simulink model "FOC"  (R2022b)
settings: Solver=FixedStepAuto  StartTime=0.0  StopTime=4  FixedStep=2e-7  RelTol=1e-3
undefined symbols (not defined in the file): sigbuilder_block
libraries: slpidlib x3, spsDCVoltageSourceLib x1, spsPermanentMagnetSynchronousMachineLib x1, simulink x1, spsUniversalBridgeLib x1, spspowerguiLib x1
settings Model: Creator=SSC  LastModifiedBy=SSC

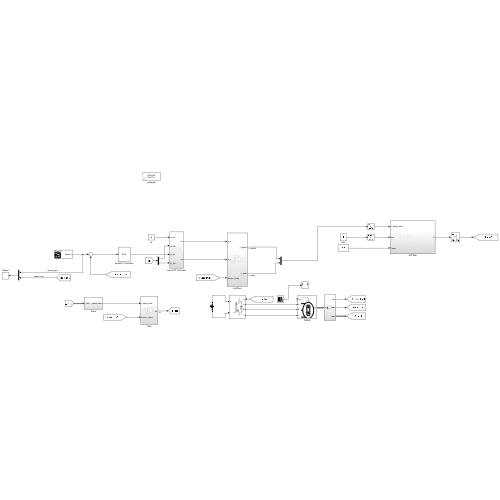
[thumbnail: Simulink's stored preview of the top-level diagram]
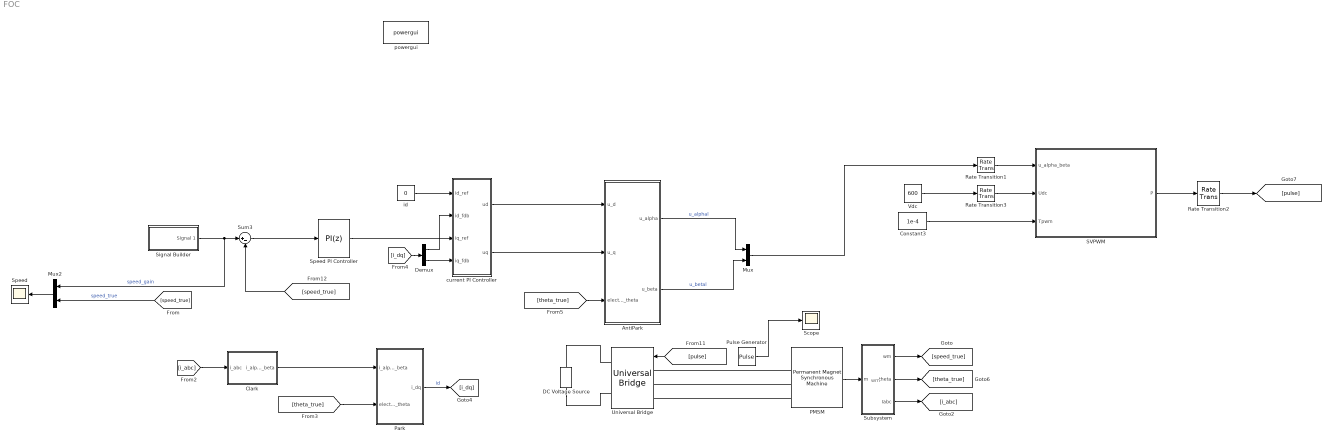
== system FOC ==
  note: wm
  AntiPark : Subsystem
  Clark : Subsystem
  Constant3 : Constant  Value=1e-4
  DC Voltage Source : spsDCVoltageSourceLib/DC Voltage Source  Amplitude=600  Measurements=None
  Demux : Demux  Outputs=2
  Mux : Mux  Inputs=2
  Mux2 : Mux  Inputs=2
  PMSM : spsPermanentMagnetSynchronousMachineLib/Permanent Magnet Synchronous Machine  NbPhases=3  FluxDistribution=Sinusoidal  RotorType=Salient-pole  MechanicalLoad=Torque Tm  PresetModel=No  ShowDetailedParameters=on  MeasurementBus=off  Resistance=0.91  Inductance=8.5e-3  dqInductances=[0.00396,0.00796]  La=8.5e-3  MachineConstant=Flux linkage established by magnets (V.s)  Flux=0.446  VoltageCst=161.7909  TorqueCst=1.338  Flat=120  Mechanical=[0.074 0.008 2 0]  PolePairs=4  InitialConditions=[0,0, 0,0]  InitialConditions5ph=[0 0 0 0 0 0]  RefAngle=Aligned with phase A axis (original Park)  IterativeDiscreteModel=Trapezoidal non iterative  TsBlock=-1  TsPowergui=0
  Park : Subsystem
  Pulse Generator : DiscretePulseGenerator  PulseType=Time based  Period=3  PulseWidth=33.3  PhaseDelay=2.5
  Rate Transition1 : RateTransition  OutPortSampleTimeOpt=Inherit
  Rate Transition2 : RateTransition
  Rate Transition3 : RateTransition  OutPortSampleTimeOpt=Inherit
  SVPWM : Subsystem
  Scope : Scope
  Signal Builder : Subsystem  Tag=STV Subsys  LoadFcn=sigbuilder_block('load');  StartFcn=sigbuilder_block('start');  StopFcn=sigbuilder_block('stop');  ClipboardFcn=sigbuilder_block('clipboard');  mask(Sigbuilder block){tuvar=[0:10]}
      mask help: Simulink:masks:SigbuilderBlock_MD
      mask init:
      | if ~strcmp(get_param(bdroot(gcbh),'SimulationStatus'),'stopped') tuvar = sigbuilder_block('maskInit'); end
      settings: CopyFcn=sigbuilder_block('copy');  DeleteFcn=sigbuilder_block('delete');  ModelCloseFcn=sigbuilder_block('modelClose');  PreSaveFcn=sigbuilder_block('preSave');  PauseFcn=sigbuilder_block('pause');  ContinueFcn=sigbuilder_block('continue');  NameChangeFcn=sigbuilder_block('namechange');  OpenFcn=sigbuilder_block('open',[290.5 134.5 550.5 400 ]);  CloseFcn=sigbuilder_block('close');
      mask Display: plot(0, 0, 100, 100,[2, 2, 32, 32, 2], [68, 8, 8, 68, 68],[32, 2], [38, 38], [32, 19, 2],[53, 60, 44], [32, 17, 17, 2],[16, 16, 31, 31]);txt = getActiveGroup(gcbh);text(2, 100, txt,'verticalAlignment', 'top');
  Speed : Scope
  Speed PI Controller : slpidlib/PID Controller  Controller=PI  Form=Parallel  TimeDomain=Discrete-time  UseExternalTs=off  SampleTime=1e-4  IntegratorMethod=Forward Euler  FilterMethod=Forward Euler  ControllerParametersSource=internal  P=3.736/30  I=44.84/30  UseKiTs=off  D=0  N=100  UseFilter=on  TunerSelectOption=Transfer Function Based (PID Tuner App)  InitialConditionSource=internal  InitialConditionForIntegrator=0  InitialConditionForFilter=0  DifferentiatorICPrevScaledInput=0  ExternalReset=none  TrackingMode=off  Kt=1  LimitOutput=off  SatLimitsSource=internal  UpperSaturationLimit=5.65  LowerSaturationLimit=-5.65  LinearizeAsGain=on  AntiWindupMode=clamping  Kb=1  LimitIntegrator=off  UpperIntegratorSaturationLimit=inf  LowerIntegratorSaturationLimit=-inf  POutMin=[]  POutMax=[]  IOutMin=[]  IOutMax=[]  DOutMin=[]  DOutMax=[]  NOutMin=[]  NOutMax=[]  SumOutMin=[]  SumOutMax=[]  SaturationOutMin=[]  SaturationOutMax=[]  PParamMin=[]  PParamMax=[]  IParamMin=[]  IParamMax=[]  DParamMin=[]  DParamMax=[]  NParamMin=[]  NParamMax=[]  KbParamMin=[]  KbParamMax=[]  KtParamMin=[]  KtParamMax=[]  KbOutMin=[]  KbOutMax=[]  KtOutMin=[]  KtOutMax=[]  IntegratorOutMin=[]  IntegratorOutMax=[]  FilterOutMin=[]  FilterOutMax=[]  SumI1OutMin=[]  SumI1OutMax=[]  SumI2OutMin=[]  SumI2OutMax=[]  SumI3OutMin=[]  SumI3OutMax=[]  SumI4OutMin=[]  SumI4OutMax=[]  SumDOutMin=[]  SumDOutMax=[]  DifferentiatorOutMin=[]  DifferentiatorOutMax=[]  FilterDiffOutCoefMin=[]  FilterDiffOutCoefMax=[]  ReciprocalOutMin=[]  ReciprocalOutMax=[]  SumDenOutMin=[]  SumDenOutMax=[]  SumNumOutMin=[]  SumNumOutMax=[]  DivideOutMin=[]  DivideOutMax=[]  UdiffTsProdOutMin=[]  UdiffTsProdOutMax=[]  NTsProdOutMin=[]  NTsProdOutMax=[]  UintegralTsProdOutMin=[]  UintegralTsProdOutMax=[]  UngainTsProdOutMin=[]  UngainTsProdOutMax=[]  ClampingZeroOutDataTypeStr=Inherit: Inherit via back propagation  ClampingZeroOutMin=[]  ClampingZeroOutMax=[]  FilterDenConstantOutDataTypeStr=Inherit: Inherit via back propagation  FilterDenConstantOutMin=[]  FilterDenConstantOutMax=[]  PCopyOutDataTypeStr=Inherit: Inherit via back propagation  PCopyOutMin=[]  PCopyOutMax=[]  NCopyOutDataTypeStr=Inherit: Inherit via back propagation  NCopyOutMin=[]  NCopyOutMax=[]  IntegratorContinuousStateAttributes=''  IntegratorStateMustResolveToSignalObject=off  IntegratorRTWStateStorageClass=Auto  FilterContinuousStateAttributes=''  FilterStateMustResolveToSignalObject=off  FilterRTWStateStorageClass=Auto  ParallelPVariant=InternalParameters  IdealPVariant=Disabled  IVariant=InternalParameters  DVariant=Disabled  IntegratorVariant=Discrete  SatVariant=Disabled  AWVariant=Passthrough  PCopyVariant=Disabled  TRVariant=Disabled  FdbkBlocksVariant=Forward  IdealPFdbkVariant=Disabled  SatFdbkVariant=Disabled  DerivativeFilterVariant=Disabled  NVariant=Disabled  NCopyVariant=Disabled_SignalSpec  FilterICVariant=Disabled  IntegratorICVariant=InternalICs  ExternalResetVariant=Disabled  TRSumVariant=Passthrough  SumFdbkVariant=Disabled  SumVariant=Sum_PI  TsampFilterVariant=InternalTs  TsampNgainVariant=Passthrough  TsampIntegralVariant=Passthrough  ExternalSaturationOutDataTypeStr=Inherit: Same as second input
  Subsystem : Subsystem
  Sum3 : Sum  Inputs=|+-
  Universal Bridge : spsUniversalBridgeLib/Universal Bridge  Arms=3  SnubberResistance=1e5  SnubberCapacitance=inf  Device=IGBT / Diodes  Ron=1e-3  Lon=0  ForwardVoltages="[  0  0  ]"  ForwardVoltage=0  GTOparameters=[ 10e-6 , 20e-6 ]  IGBTparameters=[ 1e-6 , 2e-6 ]  Measurements=None  Measurements_2=None  converterType=Rectifier
  Vdc : Constant  Value=600
  current PI Controller : Subsystem
  id : Constant  Value=0
  powergui : spspowerguiLib/powergui  Priority=1  SimulationMode=Discrete  SampleTime=2e-7  frequency=60  Iterations=50  frequencyindice=0  Pbase=100e6  ErrMax=1e-4  UnitsV=kV  UnitsW=MW  buscounter=0  FunctionMessages=off  echomessages=off  EnableUseOfTLC=off  CurrentSourceSwitches=off  DisableSnubberDevices=off  DisableRonSwitches=off  DisableVfSwitches=off  DisplayEquations=off  AutomaticDiscreteSolvers=off  SolverType=Tustin/Backward Euler (TBE)  Interpol=off  ExternalGateDelay=off  methode=off  Ts=100  x0status=blocks  SPID=on  SwTol=0  HookPort=off  NonlinearTolerance=1e-4  nMaxIteration=100  ContinueOnMaxIteration=off  RestoreLinks=warning  ResistiveCurrentMeasurement=off  Frange=[0:2:500]  Ylog=off  Xlog=on  ShowGrid=off  save=off  variable=ZData  structure=0  ZoomFFT=off  StartTime=0.0  cycles=1  DisplayStyle=1  fundamental=60  FreqAxis=off  MaxFrequency=1000  frequencyindicesteady=1  RmsSteady=1  display=off
  wires:
  [speed_true] -> Sum3/2
  Rate Transition1/1 -> SVPWM/1(u_alpha_beta)
  Demux/1 -> current PI Controller/2(id_fdb)
  Pulse Generator/1 -> Scope/1
  Speed PI Controller/1 -> current PI Controller/3(iq_ref)
  Clark/1(i_alpha_beta) -> Park/1(i_alpha_beta)
  id/1 -> current PI Controller/1(id_ref)
  [theta_true] -> Park/2(electric_theta)
  [pulse] -> Universal Bridge/1
  Demux/2 -> current PI Controller/4(iq_fdb)
  [i_dq] -> Demux/1
  Mux/1 -> Rate Transition1/1
  current PI Controller/2(uq) -> AntiPark/2(u_q)
  AntiPark/2(u_beta) -> Mux/2  "u_betal"
  Sum3/1 -> Speed PI Controller/1
  Rate Transition2/1 -> [pulse]
  Vdc/1 -> Rate Transition3/1
  Mux2/1 -> Speed/1
  Park/1(i_dq) -> [i_dq]  "id"
  Rate Transition3/1 -> SVPWM/2(Udc)
  PMSM/1 -> Subsystem/1(m)
  [theta_true] -> AntiPark/3(electric_theta)
  AntiPark/1(u_alpha) -> Mux/1  "u_alphal"
  Subsystem/1(wm) -> [speed_true]
  Constant3/1 -> SVPWM/3(Tpwm)
  Signal Builder/1(Signal 1) -> Mux2/1, Sum3/1  "speed_gain"
  current PI Controller/1(ud) -> AntiPark/1(u_d)
  Subsystem/3(Iabc) -> [i_abc]
  [speed_true] -> Mux2/2  "speed_true"
  SVPWM/1(P) -> Rate Transition2/1
  Subsystem/2(theta) -> [theta_true]
  [i_abc] -> Clark/1(i_abc)
  connections:
  Universal Bridge/RConn1 -- DC Voltage Source/RConn1
  PMSM/LConn3 -- Universal Bridge/LConn3
  DC Voltage Source/LConn1 -- Universal Bridge/RConn2
  PMSM/LConn1 -- Universal Bridge/LConn1
  PMSM/LConn2 -- Universal Bridge/LConn2

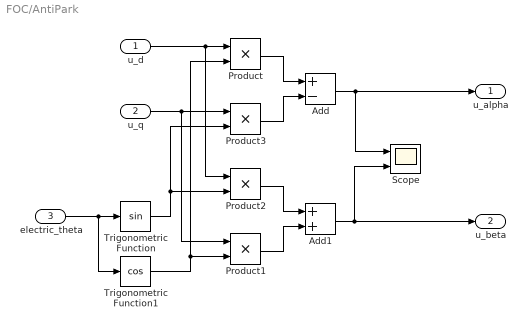
== system FOC/AntiPark ==
  u_d : Inport
  u_q : Inport  Port=2
  electric_theta : Inport  Port=3
  Add : Sum  Inputs=+-
  Add1 : Sum
  Product{,1..3} (4 alike) : Product
  Scope : Scope  NumInputPorts=2
  Trigonometric Function : Trigonometry
  Trigonometric Function1 : Trigonometry  Operator=cos
  u_alpha : Outport
  u_beta : Outport  Port=2
  wires:
  electric_theta/1 -> Trigonometric Function1/1, Trigonometric Function/1
  u_d/1 -> Product2/1, Product/1
  Trigonometric Function1/1 -> Product/2, Product1/2
  u_q/1 -> Product1/1, Product3/1
  Trigonometric Function/1 -> Product2/2, Product3/2
  Product/1 -> Add/1
  Product3/1 -> Add/2
  Add/1 -> Scope/1, u_alpha/1
  Product2/1 -> Add1/1
  Product1/1 -> Add1/2
  Add1/1 -> Scope/2, u_beta/1

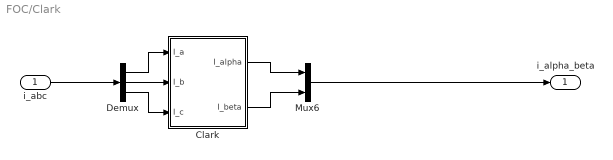
== system FOC/Clark ==
  i_abc : Inport
  Clark : Subsystem
  Demux : Demux  Outputs=3
  Mux6 : Mux  Inputs=2
  i_alpha_beta : Outport  VectorParamsAs1DForOutWhenUnconnected=off
  wires:
  Clark/2(I_beta) -> Mux6/2
  Mux6/1 -> i_alpha_beta/1
  Demux/3 -> Clark/3(I_c)
  Clark/1(I_alpha) -> Mux6/1
  i_abc/1 -> Demux/1
  Demux/2 -> Clark/2(I_b)
  Demux/1 -> Clark/1(I_a)

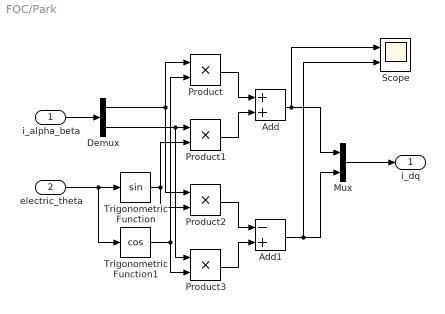
== system FOC/Park ==
  i_alpha_beta : Inport
  electric_theta : Inport  Port=2
  Add : Sum
  Add1 : Sum  Inputs=-+
  Demux : Demux  Outputs=2
  Mux : Mux  Inputs=2
  Product{,1..3} (4 alike) : Product
  Scope : Scope  NumInputPorts=2
  Trigonometric Function : Trigonometry
  Trigonometric Function1 : Trigonometry  Operator=cos
  i_dq : Outport
  wires:
  electric_theta/1 -> Trigonometric Function1/1, Trigonometric Function/1
  Trigonometric Function1/1 -> Product3/2, Product/2
  Demux/2 -> Product3/1, Product1/1
  Trigonometric Function/1 -> Product2/2, Product1/2
  Product/1 -> Add/1
  Product1/1 -> Add/2
  Product2/1 -> Add1/1
  Product3/1 -> Add1/2
  Add/1 -> Scope/1, Mux/1
  Add1/1 -> Scope/2, Mux/2
  Demux/1 -> Product/1, Product2/1
  i_alpha_beta/1 -> Demux/1
  Mux/1 -> i_dq/1

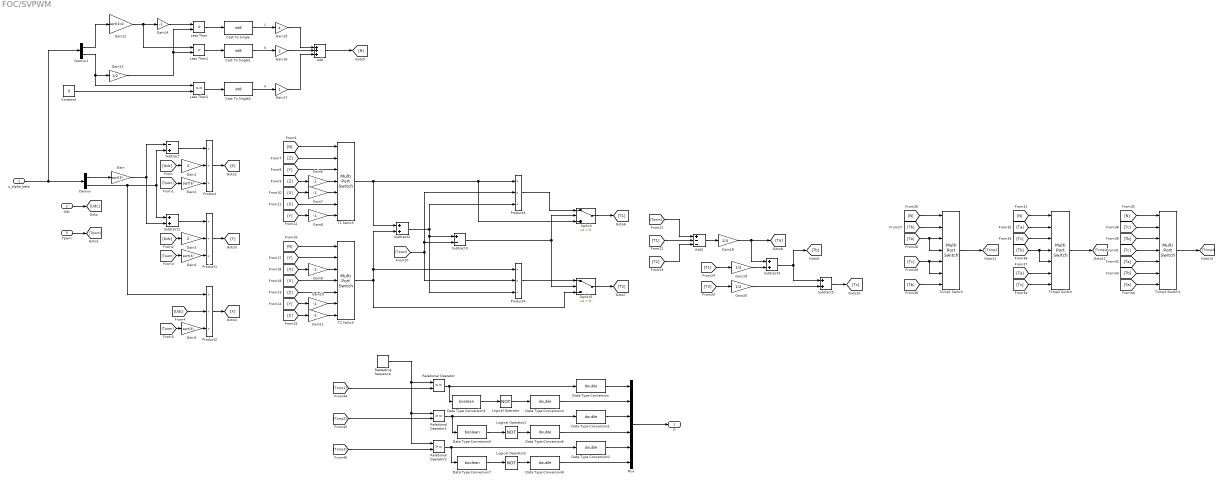
== system FOC/SVPWM ==
  u_alpha_beta : Inport
  Udc : Inport  Port=2
  Tpwm : Inport  Port=3
  Add : Sum  Inputs=+++
  Add1 : Sum  Inputs=+--
  Cast To Single : DataTypeConversion  OutDataTypeStr=int8  SaturateOnIntegerOverflow=off  RndMeth=Floor
  Cast To Single1 : DataTypeConversion  OutDataTypeStr=int8  SaturateOnIntegerOverflow=off  RndMeth=Floor
  Cast To Single2 : DataTypeConversion  OutDataTypeStr=int8  SaturateOnIntegerOverflow=off  RndMeth=Floor
  Constant : Constant  Value=0
  Data Type Conversion{,1..2,4,6,8} (6 alike) : DataTypeConversion  OutDataTypeStr=double  SaturateOnIntegerOverflow=off  RndMeth=Floor
  Data Type Conversion3 : DataTypeConversion  OutDataTypeStr=boolean  SaturateOnIntegerOverflow=off  RndMeth=Floor
  Data Type Conversion5 : DataTypeConversion  OutDataTypeStr=boolean  SaturateOnIntegerOverflow=off  RndMeth=Floor
  Data Type Conversion7 : DataTypeConversion  OutDataTypeStr=boolean  SaturateOnIntegerOverflow=off  RndMeth=Floor
  Demux : Demux  Outputs=2
  Demux1 : Demux  Outputs=2
  Gain{,2,4..5} (4 alike) : Gain  Gain=sqrt(3)
  Gain1 : Gain  Gain=2
  Gain{6..11,14} (7 alike) : Gain  Gain=-1
  Gain12 : Gain  Gain=sqrt(3)/2
  Gain13 : Gain  Gain=1/2
  Gain15 : Gain  Gain=4
  Gain16 : Gain  Gain=2
  Gain17 : Gain
  Gain18 : Gain  Gain=1/4
  Gain19 : Gain  Gain=1/2
  Gain20 : Gain  Gain=1/2
  Gain3 : Gain  Gain=2
  Less Than : RelationalOperator  Operator=>  OutDataTypeStr=boolean  RndMeth=Simplest  InputSameDT=off
  Less Than1 : RelationalOperator  Operator=>  OutDataTypeStr=boolean  RndMeth=Simplest  InputSameDT=off
  Less Than2 : RelationalOperator  OutDataTypeStr=boolean  RndMeth=Simplest  InputSameDT=off
  Logical Operator : Logic  Operator=NOT  AllPortsSameDT=off  OutDataTypeStr=boolean
  Logical Operator1 : Logic  Operator=NOT  AllPortsSameDT=off  OutDataTypeStr=boolean
  Logical Operator2 : Logic  Operator=NOT  AllPortsSameDT=off  OutDataTypeStr=boolean
  Mux : Mux  Inputs=6
  Product : Product  Inputs=*/*
  Product1 : Product  Inputs=*/*
  Product2 : Product  Inputs=*/*
  Product3 : Product  Inputs=**/
  Product4 : Product  Inputs=**/
  Relational Operator : RelationalOperator  OutDataTypeStr=boolean  RndMeth=Simplest  InputSameDT=off
  Relational Operator1 : RelationalOperator  OutDataTypeStr=boolean  RndMeth=Simplest  InputSameDT=off
  Relational Operator2 : RelationalOperator  OutDataTypeStr=boolean  RndMeth=Simplest  InputSameDT=off
  Repeating Sequence : simulink/Sources/Repeating Sequence  rep_seq_t=[0 1e-4 2e-4]  rep_seq_y=[0 0.5e-4 0]
  Subtract : Sum  Inputs=-+
  Subtract{1..2,4..5} (4 alike) : Sum
  Subtract3 : Sum  Inputs=+-
  Switch : Switch  Criteria=u2 > Threshold  SaturateOnIntegerOverflow=off  InputSameDT=off
  Switch1 : Switch  Criteria=u2 > Threshold  SaturateOnIntegerOverflow=off  InputSameDT=off
  T1 Switch : MultiPortSwitch  Inputs=6  SaturateOnIntegerOverflow=off  InputSameDT=off
  T2 Switch : MultiPortSwitch  Inputs=6  SaturateOnIntegerOverflow=off  InputSameDT=off
  Tcmp1 Switch : MultiPortSwitch  Inputs=6  SaturateOnIntegerOverflow=off  InputSameDT=off
  Tcmp2 Switch : MultiPortSwitch  Inputs=6  SaturateOnIntegerOverflow=off  InputSameDT=off
  Tcmp2 Switch1 : MultiPortSwitch  Inputs=6  SaturateOnIntegerOverflow=off  InputSameDT=off
  P : Outport
  wires:
  Demux/1 -> Gain/1
  Gain/1 -> Subtract/1, Subtract1/2
  Demux/2 -> Product2/1, Subtract/2, Subtract1/1
  Subtract/1 -> Product/1
  Udc/1 -> [Udc]
  [Udc] -> Gain1/1
  Gain1/1 -> Product/2
  Gain2/1 -> Product/3
  [Tpwm] -> Gain2/1
  Tpwm/1 -> [Tpwm]
  Product/1 -> [Z]
  Gain4/1 -> Product1/3
  [Udc] -> Gain3/1
  Gain3/1 -> Product1/2
  [Tpwm] -> Gain4/1
  Subtract1/1 -> Product1/1
  Product1/1 -> [Y]
  [Udc] -> Product2/2
  [Tpwm] -> Gain5/1
  Gain5/1 -> Product2/3
  Product2/1 -> [X]
  [N] -> T1 Switch/1
  Add/1 -> [N]
  [Z] -> T1 Switch/2
  [Y] -> T1 Switch/3
  [Z] -> Gain6/1
  [X] -> Gain7/1
  [Y] -> Gain8/1
  Gain6/1 -> T1 Switch/4
  Gain8/1 -> T1 Switch/7
  Gain7/1 -> T1 Switch/5
  [X] -> T1 Switch/6
  [X] -> T2 Switch/4
  [X] -> Gain9/1
  [Z] -> T2 Switch/5
  [N] -> T2 Switch/1
  [Y] -> T2 Switch/2
  Gain11/1 -> T2 Switch/7
  [Y] -> Gain10/1
  [Z] -> Gain11/1
  Gain9/1 -> T2 Switch/3
  Gain10/1 -> T2 Switch/6
  T1 Switch/1 -> Switch/3, Product3/1, Subtract2/1
  T2 Switch/1 -> Switch1/3, Product4/1, Subtract2/2
  Subtract2/1 -> Subtract3/1, Product4/3, Product3/3
  [Tpwm] -> Subtract3/2, Product3/2, Product4/2
  Subtract3/1 -> Switch1/2, Switch/2
  Product3/1 -> Switch/1
  Product4/1 -> Switch1/1
  Switch/1 -> [T1]
  Switch1/1 -> [T2]
  Gain16/1 -> Add/2
  u_alpha_beta/1 -> Demux1/1, Demux/1
  Gain14/1 -> Less Than/1
  Constant/1 -> Less Than2/2
  Demux1/1 -> Gain12/1
  Cast To Single2/1 -> Gain17/1  "A"
  Demux1/2 -> Gain13/1, Less Than2/1
  Less Than1/1 -> Cast To Single1/1
  Less Than2/1 -> Cast To Single2/1
  Cast To Single1/1 -> Gain16/1  "B"
  Gain17/1 -> Add/3
  Gain12/1 -> Less Than1/1, Gain14/1
  Cast To Single/1 -> Gain15/1  "C"
  Less Than/1 -> Cast To Single/1
  Gain15/1 -> Add/1
  Gain13/1 -> Less Than/2, Less Than1/2
  [Tpwm] -> Add1/1
  [T1] -> Add1/2
  [T2] -> Add1/3
  Add1/1 -> Gain18/1
  Gain18/1 -> Subtract4/1, [Ta]
  [T1] -> Gain19/1
  Gain19/1 -> Subtract4/2
  Subtract4/1 -> Subtract5/1, [Tb]
  [T2] -> Gain20/1
  Gain20/1 -> Subtract5/2
  Subtract5/1 -> [Tc]
  [N] -> Tcmp1 Switch/1
  [Tb] -> Tcmp1 Switch/2
  [Ta] -> Tcmp1 Switch/4, Tcmp1 Switch/3
  [Tc] -> Tcmp1 Switch/6, Tcmp1 Switch/5
  [Tb] -> Tcmp1 Switch/7
  Tcmp1 Switch/1 -> [Tcmp1]
  [Ta] -> Tcmp2 Switch/2
  [N] -> Tcmp2 Switch/1
  Tcmp2 Switch/1 -> [Tcmp2]
  [Tc] -> Tcmp2 Switch/3
  [Tb] -> Tcmp2 Switch/5, Tcmp2 Switch/4
  [Ta] -> Tcmp2 Switch/6
  [Tc] -> Tcmp2 Switch/7
  [Tc] -> Tcmp2 Switch1/2
  [N] -> Tcmp2 Switch1/1
  Tcmp2 Switch1/1 -> [Tcmp3]
  [Tb] -> Tcmp2 Switch1/3
  [Tc] -> Tcmp2 Switch1/4
  [Ta] -> Tcmp2 Switch1/5
  [Ta] -> Tcmp2 Switch1/7
  [Tb] -> Tcmp2 Switch1/6
  Data Type Conversion5/1 -> Logical Operator1/1
  Logical Operator/1 -> Data Type Conversion4/1
  Data Type Conversion6/1 -> Mux/4
  Logical Operator1/1 -> Data Type Conversion6/1
  Data Type Conversion4/1 -> Mux/2
  Logical Operator2/1 -> Data Type Conversion8/1
  Data Type Conversion3/1 -> Logical Operator/1
  Data Type Conversion1/1 -> Mux/3
  Data Type Conversion/1 -> Mux/1
  Data Type Conversion7/1 -> Logical Operator2/1
  Data Type Conversion8/1 -> Mux/6
  Relational Operator2/1 -> Data Type Conversion7/1, Data Type Conversion2/1
  Mux/1 -> P/1
  Data Type Conversion2/1 -> Mux/5
  [Tcmp1] -> Relational Operator/2
  [Tcmp3] -> Relational Operator2/2
  Relational Operator1/1 -> Data Type Conversion5/1, Data Type Conversion1/1
  Repeating Sequence/1 -> Relational Operator2/1, Relational Operator1/1, Relational Operator/1
  Relational Operator/1 -> Data Type Conversion3/1, Data Type Conversion/1
  [Tcmp2] -> Relational Operator1/2

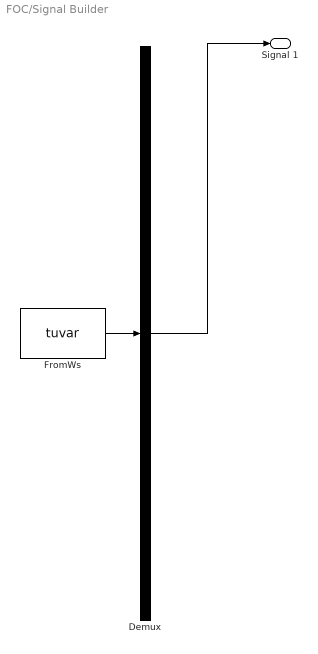
== system FOC/Signal Builder ==
  Demux : Demux  Tag=STV Demux  Outputs=1
      settings: DisplayOption=none
  FromWs : FromWorkspace  Tag=STV FromWs  VariableName=tuvar
      SigBuilderData=|
      | common.afterFinalStr = 'Extrapolate'
      | common.sampleTime = 0
      | dataSet.timeRange = [0 13]
      | dataSet.name = 'Group 1'
      | sbobj.Groups.Name = 'Group 1'
      | sbobj.Groups.Signals.Name = 'Signal 1'
      | sbobj.Groups.Signals.XData = [0 1 1.01 4 4.01 7 13]
      | sbobj.Groups.Signals.YData = [0 0 90 90 120 120 180]
      | sbobj.Groups.TimeRange = [0 13]
  Signal 1 : Outport  Tag=STV Outport
  wires:
  Demux/1 -> Signal 1/1
  FromWs/1 -> Demux/1

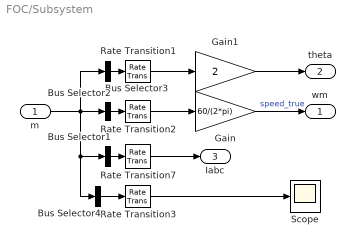
== system FOC/Subsystem ==
  m : Inport
  Bus Selector1 : BusSelector  OutputSignals=Stator current is_a (A),Stator current is_b (A),Stator current is_c (A)  OutputAsBus=on
  Bus Selector2 : BusSelector  OutputSignals=Rotor speed wm (rad/s)  OutputAsBus=on
  Bus Selector3 : BusSelector  OutputSignals=Rotor angle thetam (rad)  OutputAsBus=on
  Bus Selector4 : BusSelector  OutputSignals=Rotor speed wm (rad/s)  OutputAsBus=on
  Gain : Gain  Gain=60/(2*pi)
  Gain1 : Gain  Gain=2
  Rate Transition1 : RateTransition  OutPortSampleTime=1e-4
  Rate Transition2 : RateTransition  OutPortSampleTime=1e-4
  Rate Transition3 : RateTransition  OutPortSampleTime=1e-4
  Rate Transition7 : RateTransition
  Scope : Scope
  wm : Outport  VectorParamsAs1DForOutWhenUnconnected=off
  theta : Outport  Port=2  VectorParamsAs1DForOutWhenUnconnected=off
  Iabc : Outport  Port=3  VectorParamsAs1DForOutWhenUnconnected=off
  wires:
  Bus Selector2/1 -> Rate Transition2/1
  Bus Selector3/1 -> Rate Transition1/1
  m/1 -> Bus Selector4/1, Bus Selector1/1, Bus Selector3/1, Bus Selector2/1
  Rate Transition2/1 -> Gain/1
  Bus Selector1/1 -> Rate Transition7/1
  Rate Transition7/1 -> Iabc/1
  Rate Transition1/1 -> Gain1/1
  Bus Selector4/1 -> Rate Transition3/1
  Rate Transition3/1 -> Scope/1
  Gain/1 -> wm/1  "speed_true"
  Gain1/1 -> theta/1

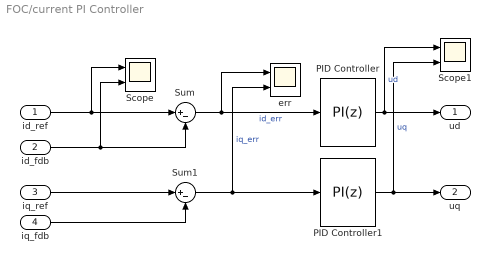
== system FOC/current PI Controller ==
  id_ref : Inport
  id_fdb : Inport  Port=2
  iq_ref : Inport  Port=3
  iq_fdb : Inport  Port=4
  PID Controller : slpidlib/PID Controller  Controller=PI  Form=Parallel  TimeDomain=Discrete-time  UseExternalTs=off  SampleTime=1e-4  IntegratorMethod=Forward Euler  FilterMethod=Forward Euler  ControllerParametersSource=internal  P=19.8  I=4550  UseKiTs=off  D=0  N=100  UseFilter=on  TunerSelectOption=Transfer Function Based (PID Tuner App)  InitialConditionSource=internal  InitialConditionForIntegrator=0  InitialConditionForFilter=0  DifferentiatorICPrevScaledInput=0  ExternalReset=none  TrackingMode=off  Kt=1  LimitOutput=on  SatLimitsSource=internal  UpperSaturationLimit=600/sqrt(3)  LowerSaturationLimit=-600/sqrt(3)  LinearizeAsGain=on  AntiWindupMode=clamping  Kb=1  LimitIntegrator=off  UpperIntegratorSaturationLimit=inf  LowerIntegratorSaturationLimit=-inf  POutMin=[]  POutMax=[]  IOutMin=[]  IOutMax=[]  DOutMin=[]  DOutMax=[]  NOutMin=[]  NOutMax=[]  SumOutMin=[]  SumOutMax=[]  SaturationOutMin=[]  SaturationOutMax=[]  PParamMin=[]  PParamMax=[]  IParamMin=[]  IParamMax=[]  DParamMin=[]  DParamMax=[]  NParamMin=[]  NParamMax=[]  KbParamMin=[]  KbParamMax=[]  KtParamMin=[]  KtParamMax=[]  KbOutMin=[]  KbOutMax=[]  KtOutMin=[]  KtOutMax=[]  IntegratorOutMin=[]  IntegratorOutMax=[]  FilterOutMin=[]  FilterOutMax=[]  SumI1OutMin=[]  SumI1OutMax=[]  SumI2OutMin=[]  SumI2OutMax=[]  SumI3OutMin=[]  SumI3OutMax=[]  SumI4OutMin=[]  SumI4OutMax=[]  SumDOutMin=[]  SumDOutMax=[]  DifferentiatorOutMin=[]  DifferentiatorOutMax=[]  FilterDiffOutCoefMin=[]  FilterDiffOutCoefMax=[]  ReciprocalOutMin=[]  ReciprocalOutMax=[]  SumDenOutMin=[]  SumDenOutMax=[]  SumNumOutMin=[]  SumNumOutMax=[]  DivideOutMin=[]  DivideOutMax=[]  UdiffTsProdOutMin=[]  UdiffTsProdOutMax=[]  NTsProdOutMin=[]  NTsProdOutMax=[]  UintegralTsProdOutMin=[]  UintegralTsProdOutMax=[]  UngainTsProdOutMin=[]  UngainTsProdOutMax=[]  ClampingZeroOutDataTypeStr=Inherit: Inherit via back propagation  ClampingZeroOutMin=[]  ClampingZeroOutMax=[]  FilterDenConstantOutDataTypeStr=Inherit: Inherit via back propagation  FilterDenConstantOutMin=[]  FilterDenConstantOutMax=[]  PCopyOutDataTypeStr=Inherit: Inherit via back propagation  PCopyOutMin=[]  PCopyOutMax=[]  NCopyOutDataTypeStr=Inherit: Inherit via back propagation  NCopyOutMin=[]  NCopyOutMax=[]  IntegratorContinuousStateAttributes=''  IntegratorStateMustResolveToSignalObject=off  IntegratorRTWStateStorageClass=Auto  FilterContinuousStateAttributes=''  FilterStateMustResolveToSignalObject=off  FilterRTWStateStorageClass=Auto  ParallelPVariant=InternalParameters  IdealPVariant=Disabled  IVariant=InternalParameters  DVariant=Disabled  IntegratorVariant=Discrete  SatVariant=Enabled  AWVariant=DiscClampingParallel  PCopyVariant=Disabled  TRVariant=Disabled  FdbkBlocksVariant=Forward  IdealPFdbkVariant=Disabled  SatFdbkVariant=Disabled  DerivativeFilterVariant=Disabled  NVariant=Disabled  NCopyVariant=Disabled_SignalSpec  FilterICVariant=Disabled  IntegratorICVariant=InternalICs  ExternalResetVariant=Disabled  TRSumVariant=Passthrough  SumFdbkVariant=Disabled  SumVariant=Sum_PI  TsampFilterVariant=InternalTs  TsampNgainVariant=Passthrough  TsampIntegralVariant=Passthrough  ExternalSaturationOutDataTypeStr=Inherit: Same as second input
  PID Controller1 : slpidlib/PID Controller  Controller=PI  Form=Parallel  TimeDomain=Discrete-time  UseExternalTs=off  SampleTime=1e-4  IntegratorMethod=Forward Euler  FilterMethod=Forward Euler  ControllerParametersSource=internal  P=19.8  I=4550  UseKiTs=off  D=0  N=100  UseFilter=on  TunerSelectOption=Transfer Function Based (PID Tuner App)  InitialConditionSource=internal  InitialConditionForIntegrator=0  InitialConditionForFilter=0  DifferentiatorICPrevScaledInput=0  ExternalReset=none  TrackingMode=off  Kt=1  LimitOutput=on  SatLimitsSource=internal  UpperSaturationLimit=600/sqrt(3)  LowerSaturationLimit=-600/sqrt(3)  LinearizeAsGain=on  AntiWindupMode=clamping  Kb=1  LimitIntegrator=off  UpperIntegratorSaturationLimit=inf  LowerIntegratorSaturationLimit=-inf  POutMin=[]  POutMax=[]  IOutMin=[]  IOutMax=[]  DOutMin=[]  DOutMax=[]  NOutMin=[]  NOutMax=[]  SumOutMin=[]  SumOutMax=[]  SaturationOutMin=[]  SaturationOutMax=[]  PParamMin=[]  PParamMax=[]  IParamMin=[]  IParamMax=[]  DParamMin=[]  DParamMax=[]  NParamMin=[]  NParamMax=[]  KbParamMin=[]  KbParamMax=[]  KtParamMin=[]  KtParamMax=[]  KbOutMin=[]  KbOutMax=[]  KtOutMin=[]  KtOutMax=[]  IntegratorOutMin=[]  IntegratorOutMax=[]  FilterOutMin=[]  FilterOutMax=[]  SumI1OutMin=[]  SumI1OutMax=[]  SumI2OutMin=[]  SumI2OutMax=[]  SumI3OutMin=[]  SumI3OutMax=[]  SumI4OutMin=[]  SumI4OutMax=[]  SumDOutMin=[]  SumDOutMax=[]  DifferentiatorOutMin=[]  DifferentiatorOutMax=[]  FilterDiffOutCoefMin=[]  FilterDiffOutCoefMax=[]  ReciprocalOutMin=[]  ReciprocalOutMax=[]  SumDenOutMin=[]  SumDenOutMax=[]  SumNumOutMin=[]  SumNumOutMax=[]  DivideOutMin=[]  DivideOutMax=[]  UdiffTsProdOutMin=[]  UdiffTsProdOutMax=[]  NTsProdOutMin=[]  NTsProdOutMax=[]  UintegralTsProdOutMin=[]  UintegralTsProdOutMax=[]  UngainTsProdOutMin=[]  UngainTsProdOutMax=[]  ClampingZeroOutDataTypeStr=Inherit: Inherit via back propagation  ClampingZeroOutMin=[]  ClampingZeroOutMax=[]  FilterDenConstantOutDataTypeStr=Inherit: Inherit via back propagation  FilterDenConstantOutMin=[]  FilterDenConstantOutMax=[]  PCopyOutDataTypeStr=Inherit: Inherit via back propagation  PCopyOutMin=[]  PCopyOutMax=[]  NCopyOutDataTypeStr=Inherit: Inherit via back propagation  NCopyOutMin=[]  NCopyOutMax=[]  IntegratorContinuousStateAttributes=''  IntegratorStateMustResolveToSignalObject=off  IntegratorRTWStateStorageClass=Auto  FilterContinuousStateAttributes=''  FilterStateMustResolveToSignalObject=off  FilterRTWStateStorageClass=Auto  ParallelPVariant=InternalParameters  IdealPVariant=Disabled  IVariant=InternalParameters  DVariant=Disabled  IntegratorVariant=Discrete  SatVariant=Enabled  AWVariant=DiscClampingParallel  PCopyVariant=Disabled  TRVariant=Disabled  FdbkBlocksVariant=Forward  IdealPFdbkVariant=Disabled  SatFdbkVariant=Disabled  DerivativeFilterVariant=Disabled  NVariant=Disabled  NCopyVariant=Disabled_SignalSpec  FilterICVariant=Disabled  IntegratorICVariant=InternalICs  ExternalResetVariant=Disabled  TRSumVariant=Passthrough  SumFdbkVariant=Disabled  SumVariant=Sum_PI  TsampFilterVariant=InternalTs  TsampNgainVariant=Passthrough  TsampIntegralVariant=Passthrough  ExternalSaturationOutDataTypeStr=Inherit: Same as second input
  Scope : Scope  NumInputPorts=2
  Scope1 : Scope  NumInputPorts=2
  Sum : Sum  Inputs=|+-
  Sum1 : Sum  Inputs=|+-
  err : Scope  NumInputPorts=2
  ud : Outport
  uq : Outport  Port=2
  wires:
  iq_fdb/1 -> Sum1/2
  Sum1/1 -> PID Controller1/1, err/2  "iq_err"
  id_fdb/1 -> Scope/2, Sum/2
  Sum/1 -> err/1, PID Controller/1  "id_err"
  id_ref/1 -> Scope/1, Sum/1
  iq_ref/1 -> Sum1/1
  PID Controller1/1 -> Scope1/2, uq/1  "uq"
  PID Controller/1 -> Scope1/1, ud/1  "ud"

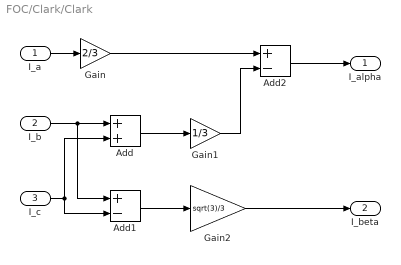
== system FOC/Clark/Clark ==
  I_a : Inport
  I_b : Inport  Port=2
  I_c : Inport  Port=3
  Add : Sum
  Add1 : Sum  Inputs=+-
  Add2 : Sum  Inputs=+-
  Gain : Gain  Gain=2/3
  Gain1 : Gain  Gain=1/3
  Gain2 : Gain  Gain=sqrt(3)/3
  I_alpha : Outport
  I_beta : Outport  Port=2
  wires:
  I_a/1 -> Gain/1
  I_b/1 -> Add1/1, Add/1
  I_c/1 -> Add/2, Add1/2
  Add/1 -> Gain1/1
  Add1/1 -> Gain2/1
  Gain/1 -> Add2/1
  Gain1/1 -> Add2/2
  Add2/1 -> I_alpha/1
  Gain2/1 -> I_beta/1
